simulink model "CartDataWriter"  (R2026b)
settings: Solver=VariableStepAuto
model mask{st=0.001, ch=1}
  mask prompts: st "Sample Time"; ch "Output Channel"
libraries: raspberrypiCommlib x1
settings Model: Creator=alex  LastModifiedBy=super

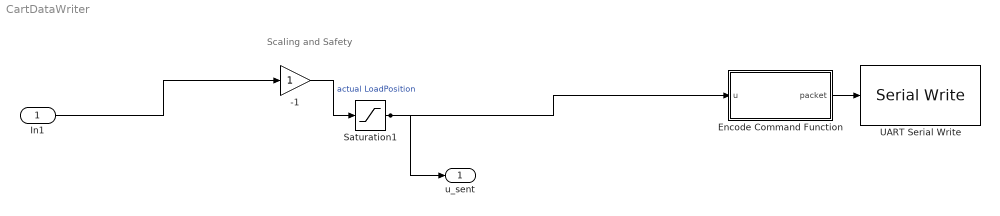
== system CartDataWriter ==
  note: Scaling and Safety
  In1 : Inport
  -1 : Gain  SaturateOnIntegerOverflow=on  OutDataTypeStr=Inherit: Same as input  ParamDataTypeStr=Inherit: Same as input
  Encode Command Function : MATLAB Function  TreatAsAtomicUnit=on
  Saturation1 : Saturate  UpperLimit=2.5  LowerLimit=-2.5
  UART Serial Write : raspberrypiCommlib/Serial Write  board=Pi 5 Model  SCIModule_=/dev/ttyAMA0  Baudrate_=230400  Parity=None  StopBits_=1  HardwareFlowControl=None  ByteOrder=LittleEndian  OutputStatus=off  blockPlatform=RaspberryPi
  u_sent : Outport
  wires:
  -1/1 -> Saturation1/1  "actual LoadPosition"
  Encode Command Function/1(packet) -> UART Serial Write/1
  In1/1 -> -1/1
  Saturation1/1 -> Encode Command Function/1(u), u_sent/1

== matlab function CartDataWriter/Encode Command Function ==
  data: u input; packet output
function packet = encode_command(u)
% Pre-allocate the exact [6x1] uint8 output array
packet = zeros(6, 1, 'uint8');

% Header bytes: 0xA5 (165), 0x5A (90)
packet(1) = uint8(165);
packet(2) = uint8(90);

% Ensure input 'u' is a scalar single (32-bit float)
u_single = single(u(1));

% Convert to 4 raw uint8 bytes (Little-Endian)
u_bytes = typecast(u_single, 'uint8');

% Explicitly assign the 4 bytes into positions 3 to 6
packet(3:6) = u_bytes(1:4);
end
